simulink library "AFCToolbox"  (R2025b)
settings: Solver=VariableStepAuto  StartTime=0.0  StopTime=10.0  RelTol=1e-3
undefined symbols (not defined in the file or in its folder): AFC5Toolbox_SimuMoudle, ax, ay, az, C_d, C_dm, C_m, C_t, Control, d, declination_table, dp0, dp1, dp2, dp3, dt, euler_0, g0, I_xyz, inclination_table, J_m, lmd_high, lmd_low, lp_acc_knoise, lp_acc_max, lp_acc_min, lp_acc_seed, lp_GPS_BL_max, lp_GPS_BL_min, lp_GPS_H_max, lp_GPS_H_min, lp_GPS_knoise, lp_GPS_seed, lp_GPS_vel_max, lp_GPS_vel_min, lp_gyro_knoise, lp_gyro_max, lp_gyro_min, lp_gyro_seed, lp_hf_vwind, lp_hs_vwind_interp, lp_kaerorho, lp_kaeroT, lp_kIxyz, lp_kmass, lp_momentx_A0, lp_momentx_Af, lp_momentx_ts, lp_momenty_A0, lp_momenty_Af, lp_momenty_ts, lp_momentz_A0, lp_momentz_Af, lp_momentz_ts, lp_vf_vwind, lp_vs_vwind_interp, lp_vwind_thetax, lp_vwind_thetaz, mass, MB_states ... (+52)
libraries: $bdroot x104, simulink x75, etargetslib x32, sharedtransform x13, simulink_extras x12, dspstat3 x11, aerolibconvert2 x9, aerolibtransform2 x3, aerolibutil x2, matrix_library x1
(part 3 of 11)

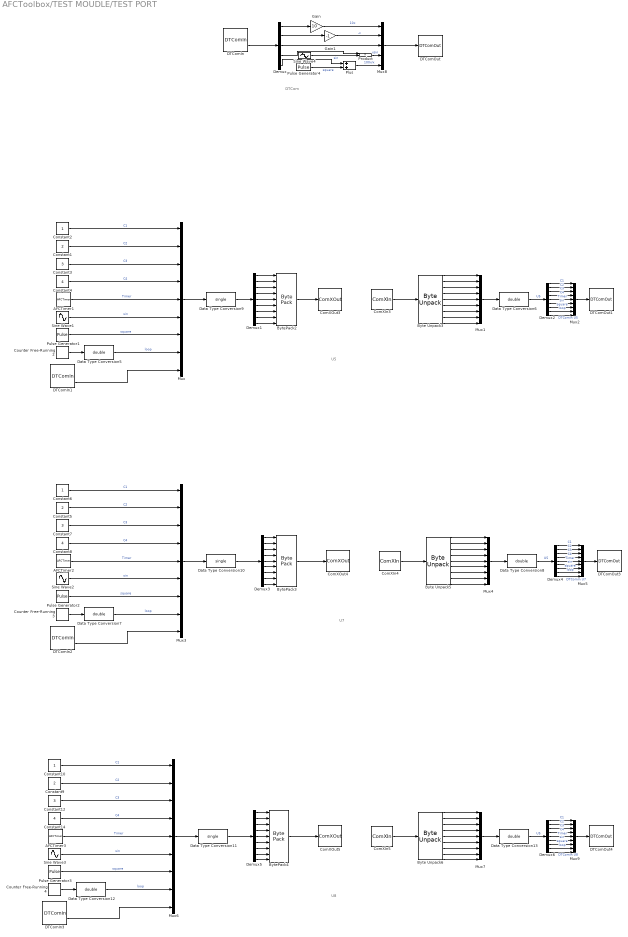
== system AFCToolbox/TEST MOUDLE/TEST PORT ==
  note: U8
  note: DTCom
  note: U7
  note: U5
  AFCTimer1 : $bdroot/DeviceModule/AFCTimer  Priority=0  g_sampleTime=0.002  g_comPort=6  g_instName=0  g_id=0
  AFCTimer2 : $bdroot/DeviceModule/AFCTimer  Priority=0  g_sampleTime=0.002  g_comPort=6  g_instName=0  g_id=0
  AFCTimer3 : $bdroot/DeviceModule/AFCTimer  Priority=0  g_sampleTime=0.002  g_comPort=6  g_instName=0  g_id=0
  Byte Unpack3 : etargetslib/Byte Unpack  dimensions={1,1,1,1,1,1,1,1,1}  datatypes={'single','single','single','single','single','single','single','single','single'}  byteAlign=1
      settings: LibrarySourceBlock=embeddedtargetslib/Host Communication/Byte Unpack
  Byte Unpack5 : etargetslib/Byte Unpack  dimensions={1,1,1,1,1,1,1,1,1}  datatypes={'single','single','single','single','single','single','single','single','single'}  byteAlign=1
      settings: LibrarySourceBlock=embeddedtargetslib/Host Communication/Byte Unpack
  Byte Unpack6 : etargetslib/Byte Unpack  dimensions={1,1,1,1,1,1,1,1,1}  datatypes={'single','single','single','single','single','single','single','single','single'}  byteAlign=1
      settings: LibrarySourceBlock=embeddedtargetslib/Host Communication/Byte Unpack
  BytePack2 : etargetslib/Byte Pack  datatypes={'single','single','single','single','single','single','single','single','single'}  byteAlign=1
  BytePack3 : etargetslib/Byte Pack  datatypes={'single','single','single','single','single','single','single','single','single'}  byteAlign=1
  BytePack4 : etargetslib/Byte Pack  datatypes={'single','single','single','single','single','single','single','single','single'}  byteAlign=1
  ComXIn3 : $bdroot/DeviceModule/ComXIn  Priority=2  g_sampleTime=0.002  g_comPort=UART5(RS422)  g_baudRate=460800  g_dataSize=36  g_parity=0  g_stopBits=1
  ComXIn4 : $bdroot/DeviceModule/ComXIn  Priority=2  g_sampleTime=0.002  g_comPort=UART7(RS232)  g_baudRate=460800  g_dataSize=36  g_parity=0  g_stopBits=1
  ComXIn5 : $bdroot/DeviceModule/ComXIn  Priority=2  g_sampleTime=0.002  g_comPort=UART8(RS232)  g_baudRate=460800  g_dataSize=36  g_parity=0  g_stopBits=1
  ComXOut3 : $bdroot/DeviceModule/ComXOut  Priority=8  g_comPort=UART5(RS422)  g_baudRate=460800  g_outFreq=10
  ComXOut4 : $bdroot/DeviceModule/ComXOut  Priority=8  g_comPort=UART7(RS232)  g_baudRate=460800  g_outFreq=10
  ComXOut5 : $bdroot/DeviceModule/ComXOut  Priority=8  g_comPort=UART8(RS232)  g_baudRate=460800  g_outFreq=10
  Constant1 : Constant  Value=2
  Constant10 : Constant
  Constant12 : Constant  Value=3
  Constant14 : Constant  Value=4
  Constant2 : Constant
  Constant3 : Constant  Value=3
  Constant4 : Constant  Value=4
  Constant5 : Constant  Value=2
  Constant6 : Constant
  Constant7 : Constant  Value=3
  Constant8 : Constant  Value=4
  Constant9 : Constant  Value=2
  Counter Free-Running2 : simulink/Sources/Counter Free-Running  NumBits=8  tsamp=-1
  Counter Free-Running3 : simulink/Sources/Counter Free-Running  NumBits=8  tsamp=-1
  Counter Free-Running4 : simulink/Sources/Counter Free-Running  NumBits=8  tsamp=-1
  DTComIn : $bdroot/DeviceModule/DTComIn  Priority=2  g_sampleTime=0.01  g_frameType=20  g_resFrameNum=0  g_comPort=6  g_instName=0  g_id=0
  DTComIn1 : $bdroot/DeviceModule/DTComIn  Priority=2  g_sampleTime=0.01  g_frameType=25  g_resFrameNum=0  g_comPort=6  g_instName=0  g_id=0
  DTComIn2 : $bdroot/DeviceModule/DTComIn  Priority=2  g_sampleTime=0.01  g_frameType=27  g_resFrameNum=0  g_comPort=6  g_instName=0  g_id=0
  DTComIn3 : $bdroot/DeviceModule/DTComIn  Priority=2  g_sampleTime=0.01  g_frameType=28  g_resFrameNum=0  g_comPort=6  g_instName=0  g_id=0
  DTComOut : $bdroot/DeviceModule/DTComOut  Priority=8  g_frameType=31  g_outFreq=1  g_comPort=0  g_instName=0  g_id=0
  DTComOut1 : $bdroot/DeviceModule/DTComOut  Priority=8  g_frameType=5  g_outFreq=10  g_comPort=0  g_instName=0  g_id=0
  DTComOut3 : $bdroot/DeviceModule/DTComOut  Priority=8  g_frameType=7  g_outFreq=10  g_comPort=0  g_instName=0  g_id=0
  DTComOut4 : $bdroot/DeviceModule/DTComOut  Priority=8  g_frameType=8  g_outFreq=10  g_comPort=0  g_instName=0  g_id=0
  Data Type Conversion10 : DataTypeConversion  OutDataTypeStr=single  SaturateOnIntegerOverflow=off  RndMeth=Floor
  Data Type Conversion11 : DataTypeConversion  OutDataTypeStr=single  SaturateOnIntegerOverflow=off  RndMeth=Floor
  Data Type Conversion{5..8,12..13} (6 alike) : DataTypeConversion  OutDataTypeStr=double  SaturateOnIntegerOverflow=off  RndMeth=Floor
  Data Type Conversion9 : DataTypeConversion  OutDataTypeStr=single  SaturateOnIntegerOverflow=off  RndMeth=Floor
  Demux : Demux  Outputs=5
  Demux{1..6} (6 alike) : Demux  Outputs=9
  Gain : Gain  Gain=10
  Gain1 : Gain  Gain=-1
  Mux{,1..7,9} (9 alike) : Mux  Inputs=9
  Mux8 : Mux  Inputs=5
  Plus : Sum
  Product : Product
  Pulse Generator{1..4} (4 alike) : DiscretePulseGenerator  PulseType=Time based  Amplitude=100  Period=1  PulseWidth=50
  Sine Wave{1..4} (4 alike) : Sin  SineType=Sample based  Samples=100  SampleTime=0.002
  wires:
  Byte Unpack6/8 -> Mux7/8
  Plus/1 -> Mux8/5  "100x/x"
  Demux6/4 -> Mux9/4  "C4"
  Data Type Conversion10/1 -> Demux3/1
  Demux/4 -> Product/1
  Demux6/6 -> Mux9/6  "sin"
  Demux3/3 -> BytePack3/3
  Demux2/9 -> Mux2/9  "DTComIn U5"
  Constant14/1 -> Mux6/4  "C4"
  Demux5/6 -> BytePack4/6
  Demux/5 -> Plus/1
  Gain/1 -> Mux8/1  "10x"
  Demux/1 -> Gain/1
  ComXIn5/1 -> Byte Unpack6/1
  Data Type Conversion13/1 -> Demux6/1  "U5"
  Data Type Conversion8/1 -> Demux4/1  "U5"
  Byte Unpack6/7 -> Mux7/7
  Sine Wave4/1 -> Product/2  "sin"
  AFCTimer1/1 -> Mux/5  "Timer"
  Pulse Generator4/1 -> Plus/2  "square"
  Byte Unpack6/9 -> Mux7/9
  Byte Unpack6/5 -> Mux7/5
  Mux8/1 -> DTComOut/1
  Byte Unpack6/1 -> Mux7/1
  Pulse Generator1/1 -> Mux/7  "square"
  Demux4/6 -> Mux5/6  "sin"
  Byte Unpack6/3 -> Mux7/3
  Byte Unpack5/9 -> Mux4/9
  Byte Unpack5/2 -> Mux4/2
  Demux5/4 -> BytePack4/4
  DTComIn/2 -> Demux/1
  Pulse Generator3/1 -> Mux6/7  "square"
  Byte Unpack3/4 -> Mux1/4
  Demux4/9 -> Mux5/9  "DTComIn U7"
  Demux6/3 -> Mux9/3  "C3"
  Mux4/1 -> Data Type Conversion8/1
  Byte Unpack6/6 -> Mux7/6
  Demux5/7 -> BytePack4/7
  Byte Unpack6/4 -> Mux7/4
  Demux2/7 -> Mux2/7  "square"
  Demux3/9 -> BytePack3/9
  Mux7/1 -> Data Type Conversion13/1
  Demux5/1 -> BytePack4/1
  Demux6/8 -> Mux9/8  "loop"
  Demux1/9 -> BytePack2/9
  Demux3/6 -> BytePack3/6
  Mux9/1 -> DTComOut4/1
  Demux6/1 -> Mux9/1  "C1"
  Demux3/4 -> BytePack3/4
  BytePack4/1 -> ComXOut5/1
  Demux6/9 -> Mux9/9  "DTComIn U8"
  AFCTimer3/1 -> Mux6/5  "Timer"
  Constant12/1 -> Mux6/3  "C3"
  Demux4/7 -> Mux5/7  "square"
  Demux6/5 -> Mux9/5  "Timer"
  Mux6/1 -> Data Type Conversion11/1
  Byte Unpack5/4 -> Mux4/4
  Demux/3 -> Mux8/3
  Demux6/2 -> Mux9/2  "C2"
  Demux2/1 -> Mux2/1  "C1"
  BytePack2/1 -> ComXOut3/1
  Data Type Conversion12/1 -> Mux6/8  "loop"
  Demux3/1 -> BytePack3/1
  Data Type Conversion11/1 -> Demux5/1
  Demux4/5 -> Mux5/5  "Timer"
  Demux3/8 -> BytePack3/8
  Demux5/8 -> BytePack4/8
  Data Type Conversion9/1 -> Demux1/1
  Demux5/5 -> BytePack4/5
  Demux/2 -> Gain1/1
  Demux6/7 -> Mux9/7  "square"
  Gain1/1 -> Mux8/2  "-x"
  Demux5/3 -> BytePack4/3
  Pulse Generator2/1 -> Mux3/7  "square"
  Demux5/2 -> BytePack4/2
  DTComIn3/2 -> Mux6/9
  Demux2/6 -> Mux2/6  "sin"
  Demux2/3 -> Mux2/3  "C3"
  Data Type Conversion6/1 -> Demux2/1  "U5"
  Byte Unpack3/8 -> Mux1/8
  Byte Unpack3/7 -> Mux1/7
  Demux3/7 -> BytePack3/7
  Sine Wave2/1 -> Mux3/6  "sin"
  Constant4/1 -> Mux/4  "C4"
  Demux1/3 -> BytePack2/3
  Demux2/4 -> Mux2/4  "C4"
  DTComIn1/2 -> Mux/9
  Counter Free-Running2/1 -> Data Type Conversion5/1
  Byte Unpack3/2 -> Mux1/2
  Sine Wave1/1 -> Mux/6  "sin"
  Constant2/1 -> Mux/1  "C1"
  Sine Wave3/1 -> Mux6/6  "sin"
  Mux2/1 -> DTComOut1/1
  Byte Unpack3/5 -> Mux1/5
  Byte Unpack3/1 -> Mux1/1
  Demux1/5 -> BytePack2/5
  Mux/1 -> Data Type Conversion9/1
  Byte Unpack3/6 -> Mux1/6
  Mux3/1 -> Data Type Conversion10/1
  Demux1/6 -> BytePack2/6
  ComXIn3/1 -> Byte Unpack3/1
  Byte Unpack3/9 -> Mux1/9
  Constant10/1 -> Mux6/1  "C1"
  Constant6/1 -> Mux3/1  "C1"
  Demux5/9 -> BytePack4/9
  Constant5/1 -> Mux3/2  "C2"
  AFCTimer2/1 -> Mux3/5  "Timer"
  Byte Unpack3/3 -> Mux1/3
  Data Type Conversion7/1 -> Mux3/8  "loop"
  Demux4/1 -> Mux5/1  "C1"
  Demux1/8 -> BytePack2/8
  Constant9/1 -> Mux6/2  "C2"
  Constant1/1 -> Mux/2  "C2"
  Mux1/1 -> Data Type Conversion6/1
  Demux4/4 -> Mux5/4  "C4"
  Demux2/2 -> Mux2/2  "C2"
  Product/1 -> Mux8/4  "xsin"
  DTComIn2/2 -> Mux3/9
  Demux2/8 -> Mux2/8  "loop"
  Demux4/8 -> Mux5/8  "loop"
  Demux3/2 -> BytePack3/2
  Demux1/4 -> BytePack2/4
  ComXIn4/1 -> Byte Unpack5/1
  BytePack3/1 -> ComXOut4/1
  Counter Free-Running3/1 -> Data Type Conversion7/1
  Byte Unpack5/1 -> Mux4/1
  Byte Unpack6/2 -> Mux7/2
  Demux1/1 -> BytePack2/1
  Byte Unpack5/3 -> Mux4/3
  Constant8/1 -> Mux3/4  "C4"
  Demux1/2 -> BytePack2/2
  Demux4/2 -> Mux5/2  "C2"
  Demux4/3 -> Mux5/3  "C3"
  Byte Unpack5/8 -> Mux4/8
  Counter Free-Running4/1 -> Data Type Conversion12/1
  Mux5/1 -> DTComOut3/1
  Constant3/1 -> Mux/3  "C3"
  Byte Unpack5/5 -> Mux4/5
  Byte Unpack5/6 -> Mux4/6
  Data Type Conversion5/1 -> Mux/8  "loop"
  Byte Unpack5/7 -> Mux4/7
  Constant7/1 -> Mux3/3  "C3"
  Demux1/7 -> BytePack2/7
  Demux2/5 -> Mux2/5  "Timer"
  Demux3/5 -> BytePack3/5

== system AFCToolbox/TEST MOUDLE/TEST PORTDOWNLOAD ==
  note: Y
  Data Type Conversion : DataTypeConversion  OutDataTypeStr=boolean  SaturateOnIntegerOverflow=off  RndMeth=Floor
  LedBit : $bdroot/DeviceModule/LedBit  Priority=6  g_chanelNo=黄色指示灯  g_comPort=0  g_instName=0  g_id=0
  Pulse Generator : DiscretePulseGenerator  PulseType=Time based  PulseWidth=50
  wires:
  Pulse Generator/1 -> Data Type Conversion/1
  Data Type Conversion/1 -> LedBit/1

== system AFCToolbox/TEST MOUDLE/TEST PWM ==
  DTComIn1 : $bdroot/DeviceModule/DTComIn  Priority=2  g_sampleTime=0.01  g_frameType=20  g_resFrameNum=0  g_comPort=6  g_instName=0  g_id=0
  DTComIn2 : $bdroot/DeviceModule/DTComIn  Priority=2  Commented=on  g_sampleTime=0.01  g_frameType=20  g_resFrameNum=0  g_comPort=6  g_instName=0  g_id=0
  DTComOut1 : $bdroot/DeviceModule/DTComOut  Priority=8  Commented=on  g_frameType=4  g_outFreq=10  g_comPort=0  g_instName=0  g_id=0
  DTComOut3 : $bdroot/DeviceModule/DTComOut  Priority=8  g_frameType=4  g_outFreq=10  g_comPort=0  g_instName=0  g_id=0
  Demux : Demux  Commented=on  Outputs=2
  Demux1 : Demux  Outputs=12
  HiEscCmd1 : $bdroot/DeviceModule/HiEscCmd  Priority=6  Commented=on  g_chanelNo=2  g_minPW=0  g_maxPW=100  g_comPort=6  g_instName=0  g_id=0
  HiEscCmd10 : $bdroot/DeviceModule/HiEscCmd  Priority=6  g_chanelNo=6  g_minPW=0  g_maxPW=100  g_comPort=6  g_instName=0  g_id=0
  HiEscCmd11 : $bdroot/DeviceModule/HiEscCmd  Priority=6  g_chanelNo=5  g_minPW=0  g_maxPW=100  g_comPort=6  g_instName=0  g_id=0
  HiEscCmd12 : $bdroot/DeviceModule/HiEscCmd  Priority=6  g_chanelNo=4  g_minPW=0  g_maxPW=100  g_comPort=6  g_instName=0  g_id=0
  HiEscCmd13 : $bdroot/DeviceModule/HiEscCmd  Priority=6  g_chanelNo=3  g_minPW=0  g_maxPW=100  g_comPort=6  g_instName=0  g_id=0
  HiEscCmd14 : $bdroot/DeviceModule/HiEscCmd  Priority=6  g_chanelNo=2  g_minPW=0  g_maxPW=100  g_comPort=6  g_instName=0  g_id=0
  HiEscCmd15 : $bdroot/DeviceModule/HiEscCmd  Priority=6  g_chanelNo=1  g_minPW=0  g_maxPW=100  g_comPort=6  g_instName=0  g_id=0
  HiEscCmd2 : $bdroot/DeviceModule/HiEscCmd  Priority=6  Commented=on  g_chanelNo=11  g_minPW=0  g_maxPW=100  g_comPort=6  g_instName=0  g_id=0
  HiEscCmd4 : $bdroot/DeviceModule/HiEscCmd  Priority=6  g_chanelNo=12  g_minPW=0  g_maxPW=100  g_comPort=6  g_instName=0  g_id=0
  HiEscCmd5 : $bdroot/DeviceModule/HiEscCmd  Priority=6  g_chanelNo=11  g_minPW=0  g_maxPW=100  g_comPort=6  g_instName=0  g_id=0
  HiEscCmd6 : $bdroot/DeviceModule/HiEscCmd  Priority=6  g_chanelNo=10  g_minPW=0  g_maxPW=100  g_comPort=6  g_instName=0  g_id=0
  HiEscCmd7 : $bdroot/DeviceModule/HiEscCmd  Priority=6  g_chanelNo=9  g_minPW=0  g_maxPW=100  g_comPort=6  g_instName=0  g_id=0
  HiEscCmd8 : $bdroot/DeviceModule/HiEscCmd  Priority=6  g_chanelNo=8  g_minPW=0  g_maxPW=100  g_comPort=6  g_instName=0  g_id=0
  HiEscCmd9 : $bdroot/DeviceModule/HiEscCmd  Priority=6  g_chanelNo=7  g_minPW=0  g_maxPW=100  g_comPort=6  g_instName=0  g_id=0
  LowEscCmd : $bdroot/DeviceModule/LowEscCmd  Priority=6  Commented=on  g_chanelNo=1  g_minPW=0  g_maxPW=100  g_comPort=6  g_instName=0  g_id=0
  LowEscCmd1 : $bdroot/DeviceModule/LowEscCmd  Priority=6  Commented=on  g_chanelNo=2  g_minPW=0  g_maxPW=100  g_comPort=6  g_instName=0  g_id=0
  LowEscCmd10 : $bdroot/DeviceModule/LowEscCmd  Priority=6  Commented=on  g_chanelNo=11  g_minPW=0  g_maxPW=100  g_comPort=6  g_instName=0  g_id=0
  LowEscCmd11 : $bdroot/DeviceModule/LowEscCmd  Priority=6  Commented=on  g_chanelNo=12  g_minPW=0  g_maxPW=100  g_comPort=6  g_instName=0  g_id=0
  LowEscCmd2 : $bdroot/DeviceModule/LowEscCmd  Priority=6  Commented=on  g_chanelNo=3  g_minPW=0  g_maxPW=100  g_comPort=6  g_instName=0  g_id=0
  LowEscCmd3 : $bdroot/DeviceModule/LowEscCmd  Priority=6  Commented=on  g_chanelNo=4  g_minPW=0  g_maxPW=100  g_comPort=6  g_instName=0  g_id=0
  LowEscCmd4 : $bdroot/DeviceModule/LowEscCmd  Priority=6  Commented=on  g_chanelNo=5  g_minPW=0  g_maxPW=100  g_comPort=6  g_instName=0  g_id=0
  LowEscCmd5 : $bdroot/DeviceModule/LowEscCmd  Priority=6  Commented=on  g_chanelNo=6  g_minPW=0  g_maxPW=100  g_comPort=6  g_instName=0  g_id=0
  LowEscCmd6 : $bdroot/DeviceModule/LowEscCmd  Priority=6  Commented=on  g_chanelNo=7  g_minPW=0  g_maxPW=100  g_comPort=6  g_instName=0  g_id=0
  LowEscCmd7 : $bdroot/DeviceModule/LowEscCmd  Priority=6  Commented=on  g_chanelNo=8  g_minPW=0  g_maxPW=100  g_comPort=6  g_instName=0  g_id=0
  LowEscCmd8 : $bdroot/DeviceModule/LowEscCmd  Priority=6  Commented=on  g_chanelNo=9  g_minPW=0  g_maxPW=100  g_comPort=6  g_instName=0  g_id=0
  LowEscCmd9 : $bdroot/DeviceModule/LowEscCmd  Priority=6  Commented=on  g_chanelNo=10  g_minPW=0  g_maxPW=100  g_comPort=6  g_instName=0  g_id=0
  Mux : Mux  Inputs=14
  Mux1 : Mux  Commented=on
  PWMSample : $bdroot/DeviceModule/PWMSample  Priority=1  g_sampleTime=0.01  g_comPort=6  g_instName=0  g_id=0
  PWMSample1 : $bdroot/DeviceModule/PWMSample  Priority=1  Commented=on  g_sampleTime=0.01  g_comPort=6  g_instName=0  g_id=0
  wires:
  PWMSample1/2 -> Mux1/4  "PWM_IN2"
  Mux1/1 -> DTComOut1/1
  Demux1/3 -> HiEscCmd13/1, Mux/3  "PWM_OUT3"
  Demux1/9 -> HiEscCmd7/1, Mux/9  "PWM_OUT9"
  Demux1/4 -> HiEscCmd12/1, Mux/4  "PWM_OUT4"
  Demux/2 -> HiEscCmd1/1, Mux1/2  "PWM_OUT12"
  Demux/1 -> HiEscCmd2/1, Mux1/1  "PWM_OUT11"
  PWMSample/2 -> Mux/14  "PWM_IN2"
  PWMSample/1 -> Mux/13  "PWM_IN1"
  Demux1/2 -> HiEscCmd14/1, Mux/2  "PWM_OUT2"
  Demux1/7 -> HiEscCmd9/1, Mux/7  "PWM_OUT7"
  Demux1/1 -> HiEscCmd15/1, Mux/1  "PWM_OUT1"
  Demux1/6 -> HiEscCmd10/1, Mux/6  "PWM_OUT6"
  Demux1/5 -> HiEscCmd11/1, Mux/5  "PWM_OUT5"
  Demux1/11 -> HiEscCmd5/1, Mux/11  "PWM_OUT11"
  Demux1/10 -> HiEscCmd6/1, Mux/10  "PWM_OUT10"
  PWMSample1/1 -> Mux1/3  "PWM_IN1"
  DTComIn1/2 -> Demux1/1
  DTComIn2/2 -> Demux/1
  Mux/1 -> DTComOut3/1
  Demux1/8 -> HiEscCmd8/1, Mux/8  "PWM_OUT8"
  Demux1/12 -> HiEscCmd4/1, Mux/12  "PWM_OUT12"

== system AFCToolbox/TEST MOUDLE/TEST SBUS ==
  note: 遥控器通讯模块
  note: PWMout
  Constant : Constant  Value=40
  Constant1 : Constant  Value=30
  Constant10 : Constant  Value=100
  Constant2 : Constant  Value=50
  Constant3 : Constant  Value=60
  Constant4 : Constant  Value=0
  Constant5 : Constant  Value=10
  Constant6 : Constant  Value=20
  Constant7 : Constant  Value=70
  Constant8 : Constant  Value=80
  Constant9 : Constant  Value=90
  DTComOut5 : $bdroot/DeviceModule/DTComOut  Priority=8  g_frameType=6  g_outFreq=10  g_comPort=0  g_instName=0  g_id=0
  HiEscCmd : $bdroot/DeviceModule/HiEscCmd  Priority=6  g_chanelNo=1  g_minPW=40  g_maxPW=80  g_comPort=6  g_instName=0  g_id=0
  HiEscCmd1 : $bdroot/DeviceModule/HiEscCmd  Priority=6  g_chanelNo=9  g_minPW=40  g_maxPW=80  g_comPort=6  g_instName=0  g_id=0
  HiEscCmd2 : $bdroot/DeviceModule/HiEscCmd  Priority=6  g_chanelNo=7  g_minPW=40  g_maxPW=80  g_comPort=6  g_instName=0  g_id=0
  HiEscCmd3 : $bdroot/DeviceModule/HiEscCmd  Priority=6  g_chanelNo=2  g_minPW=40  g_maxPW=80  g_comPort=6  g_instName=0  g_id=0
  Mux1 : Mux  Inputs=10
  SBusCmd : $bdroot/DeviceModule/SBusCmd  Priority=0  g_sampleTime=0.002  g_chanelNo=6  g_comPort=6  g_instName=0  g_id=0
  SBusCmd1 : $bdroot/DeviceModule/SBusCmd  Priority=0  g_sampleTime=0.002  g_chanelNo=1  g_comPort=6  g_instName=0  g_id=0
  SBusCmd2 : $bdroot/DeviceModule/SBusCmd  Priority=0  g_sampleTime=0.002  g_chanelNo=7  g_comPort=6  g_instName=0  g_id=0
  SBusCmd3 : $bdroot/DeviceModule/SBusCmd  Priority=0  g_sampleTime=0.002  g_chanelNo=2  g_comPort=6  g_instName=0  g_id=0
  SBusCmd4 : $bdroot/DeviceModule/SBusCmd  Priority=0  g_sampleTime=0.002  g_chanelNo=9  g_comPort=6  g_instName=0  g_id=0
  SBusCmd5 : $bdroot/DeviceModule/SBusCmd  Priority=0  g_sampleTime=0.002  g_chanelNo=3  g_comPort=6  g_instName=0  g_id=0
  SBusCmd6 : $bdroot/DeviceModule/SBusCmd  Priority=0  g_sampleTime=0.002  g_chanelNo=8  g_comPort=6  g_instName=0  g_id=0
  SBusCmd7 : $bdroot/DeviceModule/SBusCmd  Priority=0  g_sampleTime=0.002  g_chanelNo=4  g_comPort=6  g_instName=0  g_id=0
  SBusCmd8 : $bdroot/DeviceModule/SBusCmd  Priority=0  g_sampleTime=0.002  g_chanelNo=5  g_comPort=6  g_instName=0  g_id=0
  Switch{,2,5,7,9} (5 alike) : Switch  Criteria=u2 > Threshold  Threshold=1600  SaturateOnIntegerOverflow=off  InputSameDT=off
  Switch{1,3..4,6,8} (5 alike) : Switch  Criteria=u2 > Threshold  Threshold=500  SaturateOnIntegerOverflow=off  InputSameDT=off
  wires:
  Constant8/1 -> Switch7/1
  SBusCmd7/1 -> Mux1/10  "Channel4"
  Switch3/1 -> Switch/3
  SBusCmd3/1 -> Mux1/8  "Channel2"
  Switch1/1 -> Switch2/3
  SBusCmd5/1 -> Mux1/9  "Channel3"
  Constant9/1 -> Switch8/1
  Mux1/1 -> DTComOut5/1
  Switch8/1 -> Switch9/3  "pwm4"
  SBusCmd8/1 -> Mux1/1, Switch5/2, Switch4/2  "Channel5"
  Switch2/1 -> Switch6/3  "pwm4"
  SBusCmd4/1 -> Mux1/5, Switch9/2, Switch8/2  "Channel9"
  Constant6/1 -> Switch5/1
  Constant4/1 -> Switch4/3
  Switch4/1 -> Switch5/3
  Constant10/1 -> Switch9/1
  SBusCmd6/1 -> Mux1/4, Switch7/2, Switch6/2  "Channel8"
  Switch5/1 -> Switch3/3
  Constant/1 -> Switch/1
  Switch6/1 -> Switch7/3  "pwm4"
  SBusCmd1/1 -> Mux1/7  "Channel1"
  Switch/1 -> Switch1/3
  Switch9/1 -> Mux1/6, HiEscCmd/1, HiEscCmd1/1, HiEscCmd3/1, HiEscCmd2/1  "PWM"
  SBusCmd/1 -> Mux1/2, Switch/2, Switch3/2  "Channel6"
  Switch7/1 -> Switch8/3  "pwm4"
  SBusCmd2/1 -> Mux1/3, Switch1/2, Switch2/2  "Channel7"
  Constant3/1 -> Switch2/1
  Constant5/1 -> Switch4/1
  Constant1/1 -> Switch3/1
  Constant7/1 -> Switch6/1
  Constant2/1 -> Switch1/1

== system AFCToolbox/TEST MOUDLE/TEST SENSOR ==
  note: 空速计
  note: 磁力计
  note: 气压计
  DPS310 : $bdroot/DeviceModule/DPS310  Priority=1  g_sampleTime=0.01  g_comPort=6  g_instName=0  g_id=0
  DTComOut4 : $bdroot/DeviceModule/DTComOut  Priority=8  g_frameType=2  g_outFreq=10  g_comPort=0  g_instName=0  g_id=0
  IST8310 : $bdroot/DeviceModule/IST8310  Priority=1  g_sampleTime=0.01  g_comPort=0  g_instName=0  g_id=0
  MS5525 : $bdroot/DeviceModule/MS5525  Priority=1  g_sampleTime=0.01  g_comPort=6  g_instName=0  g_id=0
  Mux2 : Mux  Inputs=13
  wires:
  DPS310/1 -> Mux2/6  "Tim"
  DPS310/4 -> Mux2/9  "BarHeight"
  MS5525/2 -> Mux2/11  "IAS_DIFP"
  IST8310/5 -> Mux2/5  "HeadAng"
  IST8310/3 -> Mux2/3  "MagY"
  IST8310/4 -> Mux2/4  "MagZ"
  MS5525/1 -> Mux2/10  "IAS_TIME"
  Mux2/1 -> DTComOut4/1
  IST8310/1 -> Mux2/1  "IST_Tim"
  DPS310/2 -> Mux2/7  "Pressure"
  IST8310/2 -> Mux2/2  "agX"
  DPS310/3 -> Mux2/8  "Temprature"
  MS5525/3 -> Mux2/12  "IAS_TEMP"
  MS5525/4 -> Mux2/13  "IAS"

== system AFCToolbox/TEST MOUDLE/TEST SIMUCOM ==
  DTComOut : $bdroot/DeviceModule/DTComOut  Priority=8  g_frameType=1  g_outFreq=1  g_comPort=0  g_instName=0  g_id=0
  Demux : Demux  Outputs=8
  Mux : Mux  Inputs=8
  SimuComIn : $bdroot/DeviceModule/SimuComIn  Priority=2  g_sampleTime=0.01  g_frameType=80  g_resFrameNum=0  g_comPort=6  g_instName=0  g_id=0
  SimuComOut : $bdroot/DeviceModule/SimuComOut  Priority=8  g_frameType=1  g_outFreq=1  g_comPort=0  g_instName=0  g_id=0
  Terminator3 : Terminator
  wires:
  SimuComIn/2 -> Demux/1, SimuComOut/1
  SimuComIn/1 -> Terminator3/1
  Demux/1 -> Mux/1  "c1"
  Demux/2 -> Mux/2  "c2"
  Demux/3 -> Mux/3  "c3"
  Demux/4 -> Mux/4  "c4"
  Demux/5 -> Mux/5  "timer"
  Demux/6 -> Mux/6  "sin"
  Demux/7 -> Mux/7  "squre"
  Demux/8 -> Mux/8  "loop"
  Mux/1 -> DTComOut/1

== system AFCToolbox/TEST MOUDLE/TEST TDEBUG ==
  Data Type Conversion : DataTypeConversion  OutDataTypeStr=boolean  SaturateOnIntegerOverflow=off  RndMeth=Floor
  LedBit : $bdroot/DeviceModule/LedBit  Priority=6  g_chanelNo=蓝色指示灯  g_comPort=0  g_instName=0  g_id=0
  Pulse Generator : DiscretePulseGenerator  PulseType=Time based  PulseWidth=50
  wires:
  Pulse Generator/1 -> Data Type Conversion/1
  Data Type Conversion/1 -> LedBit/1

== system AFCToolbox/TEST MOUDLE/TSET GPS ==
  note: GPS
  DTComOut : $bdroot/DeviceModule/DTComOut  Priority=8  g_frameType=1  g_outFreq=10  g_comPort=0  g_instName=0  g_id=0
  GPS : $bdroot/DeviceModule/GPS  Priority=1  g_sampleTime=0.1  g_gpsDev=NANO GNSS  g_comPort=6  g_instName=0  g_id=0
  Mux4 : Mux  Inputs=13
  wires:
  GPS/3 -> Mux4/3  "Lat"
  GPS/13 -> Mux4/13  "AFCTim"
  GPS/1 -> Mux4/1  "GPSTim"
  GPS/10 -> Mux4/10  "Sts"
  GPS/9 -> Mux4/9  "Head"
  GPS/12 -> Mux4/12  "hdop"
  GPS/11 -> Mux4/11  "stasN"
  GPS/7 -> Mux4/7  "Vz"
  GPS/6 -> Mux4/6  "Vy"
  Mux4/1 -> DTComOut/1
  GPS/2 -> Mux4/2  "Lon"
  GPS/5 -> Mux4/5  "Vx"
  GPS/8 -> Mux4/8  "Vgnd"
  GPS/4 -> Mux4/4  "Alt"

== system AFCToolbox/基础导航算法模型库/ECL EKF ==
  note: EKF2.cpp -> Run(...)
  note: 2024.03.28午3时半：
      | 整理的新版本EKF导航（single型），包括磁力计、气压计、GPS融合数仿程序
  note: headang
  gyro(rad/s) : Inport
  acc(m2/s) : Inport  Port=2
  Vgps(m/s) : Inport  Port=3
  LLA(deg) : Inport  Port=4
  Gps_sts : Inport  Port=5
  Magxyz(uT) : Inport  Port=6
  BARO_Data(Pa) : Inport  Port=7
  Tim : Inport  Port=8
  Bias Eliminate2 : Subsystem
  Bus Creator : BusCreator  Inputs=q_states(1:4),Vned_states(5:7),Pned_states(8:10),Δθb_states(11:13),ΔVb_states(14:16),MI_states(17:19),MB_states(20:22),Vwind_states(23:24)
  Constant : Constant  Value=[-19.98,-8.18,31.27]
  Data Type Conversion{1,6..8} (4 alike) : DataTypeConversion  OutDataTypeStr=double  SaturateOnIntegerOverflow=off  RndMeth=Floor
  Data Type Conversion{2..5} (4 alike) : DataTypeConversion  OutDataTypeStr=single  SaturateOnIntegerOverflow=off  RndMeth=Floor
  Demux1 : Demux  Outputs=3
  Gain : Gain  Gain=0.01
  Gain10 : Gain  Gain=1/57.3
  Gain11 : Gain  Gain=1/57.3
  Gain12 : Gain
  Gain6 : Gain  Gain=dt
  Gain7 : Gain  Gain=dt
  Gain9 : Gain
  Mux12 : Mux  Inputs=3
  Subsystem : Subsystem
  Subsystem1 : Subsystem
  Subsystem2 : Subsystem
  Subtract : Sum
  Tim1 : InportShadow  Port=8
  Zero-Order Hold10 : ZeroOrderHold  SampleTime=-1
  Zero-Order Hold2 : ZeroOrderHold  SampleTime=dt
  Zero-Order Hold5 : ZeroOrderHold  SampleTime=-1
  Zero-Order Hold8 : ZeroOrderHold  SampleTime=dt
  Zero-Order Hold9 : ZeroOrderHold  SampleTime=-1
  init_state : Subsystem
  states(11:13) : Constant  Value=zeros(1,3)  OutDataTypeStr=single
  states(14:16) : Constant  Value=zeros(1,3)  OutDataTypeStr=single
  states(20:22) : Constant  Value=zeros(1,3)  OutDataTypeStr=single
  states(23:24) : Constant  Value=zeros(1,2)  OutDataTypeStr=single
  ekf_psithephi : Outport
  ekf_xyz : Outport  Port=2
  gps : Outport  Port=3
  Pned : Outport  Port=4
  wires:
  Subtract/1 -> Zero-Order Hold8/1
  Magxyz(uT)/1 -> Subtract/1
  Tim1/1 -> Subsystem1/2(In2)
  Tim/1 -> Subsystem2/2(Tim)
  Demux1/2 -> Gain11/1
  Zero-Order Hold10/1 -> Data Type Conversion5/1
  init_state/3(states(8:10)) -> Bus Creator/3, Data Type Conversion1/1  "Pned_states(8:10)"
  states(14:16)/1 -> Bus Creator/5  "ΔVb_states(14:16)"
  acc(m2/s)/1 -> Zero-Order Hold10/1
  init_state/2(states(5:7)) -> Bus Creator/2  "Vned_states(5:7)"
  states(11:13)/1 -> Bus Creator/4  "Δθb_states(11:13)"
  LLA(deg)/1 -> Data Type Conversion8/1
  Data Type Conversion3/1 -> Bias Eliminate2/1(gyro_B_rad/s_ori)  "gyro_B_rad/s_LPF"
  Zero-Order Hold2/1 -> Data Type Conversion6/1
  Data Type Conversion1/1 -> Pned/1
  init_state/6(Mag_sensordata) -> Subsystem/5(Mag_sensordta)  "Mag_sensordta"
  Subsystem/2(p_ekfnew) -> ekf_xyz/1  "ekf_xyz"
  states(23:24)/1 -> Bus Creator/8  "Vwind_states(23:24)"
  Subsystem/3(GPS_xyz) -> gps/1  "gps"
  Zero-Order Hold5/1 -> init_state/7(baro_data_p)  "BARO_Data"
  Data Type Conversion5/1 -> Gain7/1
  Subsystem/1(ekf_new) -> ekf_psithephi/1  "ekf_psithephi"
  Gain9/1 -> Zero-Order Hold2/1
  Constant/1 -> Subtract/2
  Bias Eliminate2/1(Out1) -> Zero-Order Hold9/1  "gyro_B_rad/s_LPF"
  Vgps(m/s)/1 -> Gain9/1
  Demux1/3 -> Gain12/1
  Data Type Conversion4/1 -> Gain6/1
  Subsystem2/1(enable) -> init_state/6(QGC_sensor_reinit)
  Data Type Conversion8/1 -> Demux1/1
  Subsystem1/1(enable) -> Subsystem/Enable
  Zero-Order Hold8/1 -> Data Type Conversion2/1
  init_state/5(BARO_Data) -> Subsystem/4(BARO_Data)  "BARO_Data"
  Mux12/1 -> init_state/3(gps_LLA_rad)
  Zero-Order Hold9/1 -> Data Type Conversion4/1
  Data Type Conversion2/1 -> Gain/1
  Gain/1 -> init_state/8(mag)  "Guass"
  Data Type Conversion6/1 -> init_state/4(GPS_Vecef_m/s)
  gyro(rad/s)/1 -> Data Type Conversion3/1
  BARO_Data(Pa)/1 -> Zero-Order Hold5/1
  Data Type Conversion7/1 -> init_state/5(GPSfixtype)
  init_state/7(GPS_sensordata) -> Subsystem/6(GPS_sensordata)  "GPS_sensordata"
  Gain10/1 -> Mux12/1
  Gain11/1 -> Mux12/2
  Gain7/1 -> Subsystem/2(imu_delta_vel), init_state/2(imu_data_del_vel)
  Bus Creator/1 -> Subsystem/3(init_states)  "init_states"
  Gain6/1 -> Subsystem/1(imu_delta_angle), init_state/1(imu_delta_ang)
  ? -> init_state/9(states)
  Demux1/1 -> Gain10/1
  init_state/4(states(17:19)) -> Bus Creator/6  "MI_states(17:19)"
  init_state/1(states(1:4)) -> Bus Creator/1  "q_states(1:4)"
  states(20:22)/1 -> Bus Creator/7  "MB_states(20:22)"
  Gain12/1 -> Mux12/3
  Gps_sts/1 -> Subsystem1/1(Gps_sts), Data Type Conversion7/1, Subsystem2/1(Gps_sts)

== system AFCToolbox/ServoCardModule/XSimPack/ByteCheckSum ==
  In1 : Inport
  Add : Sum
  Bitwise AND : simulink/Logic and Bit Operations/Bitwise Operator  logicop=AND  UseBitMask=on  BitMask=hex2dec('FF')  BitMaskRealWorld=Stored Integer
      settings: LibrarySourceBlock=|
      | simulink/Quick Insert/Logic and Bit
      | Operations/Bitwise AND
  Bitwise AND1 : simulink/Logic and Bit Operations/Bitwise Operator  logicop=AND  UseBitMask=on  BitMask=hex2dec('FF')  BitMaskRealWorld=Stored Integer
      settings: LibrarySourceBlock=|
      | simulink/Quick Insert/Logic and Bit
      | Operations/Bitwise AND
  Bitwise NOT : simulink/Logic and Bit Operations/Bitwise Operator  logicop=NOT  UseBitMask=off  BitMask=bin2dec('11011001')  BitMaskRealWorld=Stored Integer
      settings: LibrarySourceBlock=|
      | simulink/Quick Insert/Logic and Bit
      | Operations/Bitwise NOT
  Constant5 : Constant
  Data Type Conversion10 : DataTypeConversion  OutDataTypeStr=uint8  SaturateOnIntegerOverflow=off  RndMeth=Floor
  Data Type Conversion11 : DataTypeConversion  OutDataTypeStr=uint16  SaturateOnIntegerOverflow=off  RndMeth=Floor
  Data Type Conversion12 : DataTypeConversion  OutDataTypeStr=uint8  SaturateOnIntegerOverflow=off  RndMeth=Floor
  Data Type Conversion8 : DataTypeConversion  OutDataTypeStr=uint32  SaturateOnIntegerOverflow=off  RndMeth=Floor
  Data Type Conversion9 : DataTypeConversion  OutDataTypeStr=uint16  SaturateOnIntegerOverflow=off  RndMeth=Floor
  Sum of Elements : Sum  Inputs=+
  Out1 : Outport
  wires:
  Bitwise NOT/1 -> Data Type Conversion9/1
  Constant5/1 -> Data Type Conversion11/1
  Sum of Elements/1 -> Bitwise AND/1
  Bitwise AND/1 -> Data Type Conversion10/1
  Add/1 -> Bitwise AND1/1
  Data Type Conversion9/1 -> Add/1
  Data Type Conversion11/1 -> Add/2
  Data Type Conversion8/1 -> Sum of Elements/1
  Data Type Conversion10/1 -> Bitwise NOT/1
  In1/1 -> Data Type Conversion8/1
  Data Type Conversion12/1 -> Out1/1
  Bitwise AND1/1 -> Data Type Conversion12/1

== system AFCToolbox/ServoCardModule/XSimUnPack/FrameCheck ==
  note: 判断前两个字节帧头、次两个字节帧长度、校验和
  In1 : Inport
  AND : Logic  Inputs=3  IconShape=distinctive  AllPortsSameDT=off  OutDataTypeStr=boolean
  Bitwise AND : simulink/Logic and Bit Operations/Bitwise Operator  logicop=AND  UseBitMask=on  BitMask=hex2dec('FF')  BitMaskRealWorld=Stored Integer
      settings: LibrarySourceBlock=|
      | simulink/Quick Insert/Logic and Bit
      | Operations/Bitwise AND
  Byte Unpack1 : etargetslib/Byte Unpack  dimensions={1}  datatypes={'uint16'}  byteAlign=1
      settings: LibrarySourceBlock=embeddedtargetslib/Host Communication/Byte Unpack
  Byte Unpack3 : etargetslib/Byte Unpack  dimensions={1}  datatypes={'uint16'}  byteAlign=1
      settings: LibrarySourceBlock=embeddedtargetslib/Host Communication/Byte Unpack
  Compare To Constant : simulink/Logic and Bit Operations/Compare To Constant  relop===  const=hex2dec('DAA5')  OutDataTypeStr=boolean
  Compare To Zero : simulink/Logic and Bit Operations/Compare To Zero  relop===  OutDataTypeStr=boolean
  Data Type Conversion : DataTypeConversion  OutDataTypeStr=uint32  SaturateOnIntegerOverflow=off  RndMeth=Floor
  Data Type Conversion1 : DataTypeConversion  OutDataTypeStr=uint8  SaturateOnIntegerOverflow=off  RndMeth=Floor
  Demux : Demux  Outputs=[2,2,-1]
      settings: DisplayOption=none
  Relational Operator : RelationalOperator  Operator===  OutDataTypeStr=boolean  RndMeth=Simplest  InputSameDT=off
  Sum ofElements : Sum  Inputs=+
  Terminator : Terminator
  Width : Width  DataType=uint16
  Out1 : Outport
  wires:
  AND/1 -> Out1/1
  Bitwise AND/1 -> Data Type Conversion1/1
  Demux/1 -> Byte Unpack3/1
  Compare To Constant/1 -> AND/1
  Compare To Zero/1 -> AND/3
  Width/1 -> Relational Operator/2
  Relational Operator/1 -> AND/2
  Demux/2 -> Byte Unpack1/1
  Byte Unpack1/1 -> Relational Operator/1
  In1/1 -> Demux/1, Data Type Conversion/1, Width/1
  Data Type Conversion/1 -> Sum ofElements/1
  Byte Unpack3/1 -> Compare To Constant/1
  Demux/3 -> Terminator/1
  Data Type Conversion1/1 -> Compare To Zero/1
  Sum ofElements/1 -> Bitwise AND/1

== system AFCToolbox/ServoCardModule/XSimUnPack/Subsystem2 ==
  note: 除去帧头等12个字节之外的数据字节长度，如果为4的倍数则正常并解析为单精度，否则不进行解析（强行解析后报错）
  Frame : Inport
  Enable : EnablePort
  Byte Unpack3 : etargetslib/Byte Unpack  dimensions={1}  datatypes={'uint32'}  byteAlign=1
      settings: LibrarySourceBlock=embeddedtargetslib/Host Communication/Byte Unpack
  Compare To Zero : simulink/Logic and Bit Operations/Compare To Zero  relop===  OutDataTypeStr=boolean
  Constant : Constant  Value=4  OutDataTypeStr=uint16
  Data Type Conversion{,1..4} (5 alike) : DataTypeConversion  OutDataTypeStr=double  SaturateOnIntegerOverflow=off  RndMeth=Floor
  Demux : Demux  Outputs=[2,2,4,1,1,1,-1,1]
      settings: DisplayOption=none
  Mod : Math  Operator=mod
  Subsystem : Subsystem
  Terminator : Terminator
  Terminator1 : Terminator
  Terminator2 : Terminator
  Width : Width  DataType=uint16
  FrameCounter : Outport
  SourceID : Outport  Port=2
  TargetID : Outport  Port=3
  FrameType : Outport  Port=4
  FramePara : Outport  Port=5
  wires:
  Constant/1 -> Mod/2
  Data Type Conversion3/1 -> TargetID/1
  Demux/4 -> Data Type Conversion2/1
  Frame/1 -> Demux/1
  Demux/8 -> Terminator/1
  Width/1 -> Mod/1
  Byte Unpack3/1 -> Data Type Conversion1/1
  Demux/3 -> Byte Unpack3/1
  Data Type Conversion4/1 -> FrameType/1
  Data Type Conversion1/1 -> FrameCounter/1
  Demux/6 -> Data Type Conversion4/1
  Demux/5 -> Data Type Conversion3/1
  Demux/2 -> Terminator1/1
  Demux/7 -> Subsystem/1(In1), Width/1
  Data Type Conversion2/1 -> SourceID/1
  Demux/1 -> Terminator2/1
  Subsystem/1(Out1) -> Data Type Conversion/1
  Data Type Conversion/1 -> FramePara/1
  Mod/1 -> Compare To Zero/1
  Compare To Zero/1 -> Subsystem/Enable

== system AFCToolbox/ServoCardModule/XSrvoCmd/查询四个舵机角度指令 ==
  note: 查询四个舵机的角度信息
  note: 长度
  note: 读取数据长度
  Bitwise AND : simulink/Logic and Bit Operations/Bitwise Operator  logicop=AND  UseBitMask=on  BitMask=0xFF  BitMaskRealWorld=Stored Integer
      settings: LibrarySourceBlock=|
      | simulink/Quick Insert/Logic and Bit
      | Operations/Bitwise AND
  Bitwise NOT : simulink/Logic and Bit Operations/Bitwise Operator  logicop=NOT  UseBitMask=off  BitMask=bin2dec('11011001')  BitMaskRealWorld=Stored Integer
      settings: LibrarySourceBlock=|
      | simulink/Quick Insert/Logic and Bit
      | Operations/Bitwise NOT
  Constant10 : Constant  Value=0x38  OutDataTypeStr=uint8
  Constant11 : Constant  Value=0x02  OutDataTypeStr=uint8
  Constant12 : Constant  Value=0xFF  OutDataTypeStr=uint8
  Constant13 : Constant  Value=0x01
  Constant14 : Constant  Value=0x03
  Constant15 : Constant  Value=0x02
  Constant16 : Constant  Value=0x04
  Constant17 : Constant  Value=0x08  OutDataTypeStr=uint8
  Constant6 : Constant  Value=0xFF  OutDataTypeStr=uint8
  Constant7 : Constant  Value=0xFE  OutDataTypeStr=uint8
  Constant9 : Constant  Value=0x82  OutDataTypeStr=uint8
  Data Type Conversion : DataTypeConversion  OutDataTypeStr=uint32  SaturateOnIntegerOverflow=off  RndMeth=Floor
  Data Type Conversion1 : DataTypeConversion  OutDataTypeStr=uint8  SaturateOnIntegerOverflow=off  RndMeth=Floor
  Mux2 : Mux
  Mux3 : Mux  Inputs=9
  Sum ofElements : Sum  Inputs=+
  RAng : Outport
  wires:
  Constant16/1 -> Mux3/9
  Mux3/1 -> Data Type Conversion/1, Mux2/3
  Bitwise AND/1 -> Data Type Conversion1/1
  Data Type Conversion1/1 -> Bitwise NOT/1
  Constant17/1 -> Mux3/2
  Mux2/1 -> RAng/1
  Constant12/1 -> Mux2/2
  Data Type Conversion/1 -> Sum ofElements/1
  Sum ofElements/1 -> Bitwise AND/1
  Constant14/1 -> Mux3/8
  Constant6/1 -> Mux2/1
  Constant13/1 -> Mux3/6
  Constant15/1 -> Mux3/7
  Constant10/1 -> Mux3/4
  Constant11/1 -> Mux3/5
  Bitwise NOT/1 -> Mux2/4
  Constant7/1 -> Mux3/1
  Constant9/1 -> Mux3/3

== system AFCToolbox/ServoCardModule/XSrvoCmd/设置四个舵机位置与速度指令 ==
  Ang : Inport
  Byte Pack : etargetslib/Byte Pack  datatypes={'uint8','uint8','uint8','uint8','uint8','uint8','uint8'}  byteAlign=1
  Constant : Constant  Value=0xFF  OutDataTypeStr=uint8
  Constant1 : Constant  Value=0xFF  OutDataTypeStr=uint8
  Constant2 : Constant  Value=0x20  OutDataTypeStr=uint8
  Constant3 : Constant  Value=0x83  OutDataTypeStr=uint8
  Constant4 : Constant  Value=0x2A  OutDataTypeStr=uint8
  Constant5 : Constant  Value=0x06  OutDataTypeStr=uint8
  Constant6 : Constant  Value=180
  Constant8 : Constant  Value=0xFE  OutDataTypeStr=uint8
  Demux : Demux
  GetCheckSum2 : Subsystem
  Mux : Mux  Inputs=2
  Mux1 : Mux  Inputs=5
  Subsystem1 : Subsystem  mask{id=2}
      mask DialogControl ParameterGroupVar Prompt: id
  Subsystem2 : Subsystem  mask{id=3}
      mask DialogControl ParameterGroupVar Prompt: id
  Subsystem3 : Subsystem  mask{id=4}
      mask DialogControl ParameterGroupVar Prompt: id
  Subsystem5 : Subsystem  mask{id=1}
      mask DialogControl ParameterGroupVar Prompt: id
  Subtract{,1..3} (4 alike) : Sum
  Frame : Outport
  wires:
  Mux/1 -> Frame/1
  Constant4/1 -> Byte Pack/6
  Mux1/1 -> Mux/1, GetCheckSum2/1(In1)
  GetCheckSum2/1(Out1) -> Mux/2
  Constant5/1 -> Byte Pack/7
  Constant2/1 -> Byte Pack/4
  Constant1/1 -> Byte Pack/2
  Constant/1 -> Byte Pack/1
  Constant3/1 -> Byte Pack/5
  Constant8/1 -> Byte Pack/3
  Byte Pack/1 -> Mux1/1
  Demux/3 -> Subtract2/1
  Subtract2/1 -> Subsystem2/1(p)
  Subtract3/1 -> Subsystem3/1(p)
  Ang/1 -> Demux/1
  Demux/1 -> Subtract/1
  Constant6/1 -> Subtract3/2, Subtract2/2, Subtract1/2, Subtract/2
  Subtract1/1 -> Subsystem1/1(p)
  Subtract/1 -> Subsystem5/1(p)
  Demux/2 -> Subtract1/1
  Demux/4 -> Subtract3/1
  Subsystem5/1(Out1) -> Mux1/2
  Subsystem1/1(Out1) -> Mux1/3
  Subsystem2/1(Out1) -> Mux1/4
  Subsystem3/1(Out1) -> Mux1/5

== system AFCToolbox/ServoCardModule/XSrvoSamp/SrvoPro ==
  SvoFrame : Inport
  AND1 : Logic  Inputs=4  IconShape=distinctive  AllPortsSameDT=off  OutDataTypeStr=boolean
  Bitwise AND4 : simulink/Logic and Bit Operations/Bitwise Operator  logicop=AND  UseBitMask=on  BitMask=hex2dec('FF')  BitMaskRealWorld=Stored Integer
      settings: LibrarySourceBlock=|
      | simulink/Quick Insert/Logic and Bit
      | Operations/Bitwise AND
  Byte Unpack4 : etargetslib/Byte Unpack  dimensions={[1]}  datatypes={'uint16'}  byteAlign=1
      settings: LibrarySourceBlock=embeddedtargetslib/Host Communication/Byte Unpack
  Compare To Constant1 : simulink/Logic and Bit Operations/Compare To Constant  relop===  const=0xFF  OutDataTypeStr=boolean
  Compare To Constant2 : simulink/Logic and Bit Operations/Compare To Constant  relop===  const=0x00  OutDataTypeStr=boolean
  Compare To Constant8 : simulink/Logic and Bit Operations/Compare To Constant  relop===  const=0xFFFF  OutDataTypeStr=boolean
  Compare To Constant9 : simulink/Logic and Bit Operations/Compare To Constant  relop===  const=0x04  OutDataTypeStr=boolean
  Data Type Conversion8 : DataTypeConversion  OutDataTypeStr=uint32  SaturateOnIntegerOverflow=off  RndMeth=Floor
  Data Type Conversion9 : DataTypeConversion  OutDataTypeStr=uint8  SaturateOnIntegerOverflow=off  RndMeth=Floor
  Demux : Demux  Outputs=[2,1,1,1,2,1]
  Mux : Mux  Inputs=5
  Subsystem : Subsystem
  Sum ofElements4 : Sum  Inputs=+
  ID : Outport
  angleACK : Outport  Port=2
  wires:
  AND1/1 -> Subsystem/Enable
  Demux/6 -> Mux/5  "CHK"
  Subsystem/1(Outport) -> angleACK/1
  Demux/5 -> Subsystem/1(In1), Mux/4  "POS"
  Demux/3 -> Mux/2, Compare To Constant9/1  "LEN"
  Compare To Constant2/1 -> AND1/3
  Demux/2 -> ID/1, Mux/1  "ID"
  Data Type Conversion8/1 -> Sum ofElements4/1
  Compare To Constant9/1 -> AND1/2
  Sum ofElements4/1 -> Bitwise AND4/1
  Demux/4 -> Compare To Constant2/1, Mux/3  "STS"
  Byte Unpack4/1 -> Compare To Constant8/1
  Mux/1 -> Data Type Conversion8/1
  Compare To Constant8/1 -> AND1/1
  Data Type Conversion9/1 -> Compare To Constant1/1
  Bitwise AND4/1 -> Data Type Conversion9/1
  Demux/1 -> Byte Unpack4/1  "FrameHead"
  Compare To Constant1/1 -> AND1/4
  SvoFrame/1 -> Demux/1

== system AFCToolbox/ServoCardModule/XSrvoSamp/SrvoPro1 ==
  SvoFrame : Inport
  AND1 : Logic  Inputs=4  IconShape=distinctive  AllPortsSameDT=off  OutDataTypeStr=boolean
  Bitwise AND4 : simulink/Logic and Bit Operations/Bitwise Operator  logicop=AND  UseBitMask=on  BitMask=hex2dec('FF')  BitMaskRealWorld=Stored Integer
      settings: LibrarySourceBlock=|
      | simulink/Quick Insert/Logic and Bit
      | Operations/Bitwise AND
  Byte Unpack4 : etargetslib/Byte Unpack  dimensions={[1]}  datatypes={'uint16'}  byteAlign=1
      settings: LibrarySourceBlock=embeddedtargetslib/Host Communication/Byte Unpack
  Compare To Constant1 : simulink/Logic and Bit Operations/Compare To Constant  relop===  const=0xFF  OutDataTypeStr=boolean
  Compare To Constant2 : simulink/Logic and Bit Operations/Compare To Constant  relop===  const=0x00  OutDataTypeStr=boolean
  Compare To Constant8 : simulink/Logic and Bit Operations/Compare To Constant  relop===  const=0xFFFF  OutDataTypeStr=boolean
  Compare To Constant9 : simulink/Logic and Bit Operations/Compare To Constant  relop===  const=0x04  OutDataTypeStr=boolean
  Data Type Conversion8 : DataTypeConversion  OutDataTypeStr=uint32  SaturateOnIntegerOverflow=off  RndMeth=Floor
  Data Type Conversion9 : DataTypeConversion  OutDataTypeStr=uint8  SaturateOnIntegerOverflow=off  RndMeth=Floor
  Demux : Demux  Outputs=[2,1,1,1,2,1]
  Mux : Mux  Inputs=5
  Subsystem : Subsystem
  Sum ofElements4 : Sum  Inputs=+
  ID : Outport
  angleACK : Outport  Port=2
  wires:
  AND1/1 -> Subsystem/Enable
  Demux/6 -> Mux/5  "CHK"
  Subsystem/1(Outport) -> angleACK/1
  Demux/5 -> Subsystem/1(In1), Mux/4  "POS"
  Demux/3 -> Mux/2, Compare To Constant9/1  "LEN"
  Compare To Constant2/1 -> AND1/3
  Demux/2 -> ID/1, Mux/1  "ID"
  Data Type Conversion8/1 -> Sum ofElements4/1
  Compare To Constant9/1 -> AND1/2
  Sum ofElements4/1 -> Bitwise AND4/1
  Demux/4 -> Compare To Constant2/1, Mux/3  "STS"
  Byte Unpack4/1 -> Compare To Constant8/1
  Mux/1 -> Data Type Conversion8/1
  Compare To Constant8/1 -> AND1/1
  Data Type Conversion9/1 -> Compare To Constant1/1
  Bitwise AND4/1 -> Data Type Conversion9/1
  Demux/1 -> Byte Unpack4/1  "FrameHead"
  Compare To Constant1/1 -> AND1/4
  SvoFrame/1 -> Demux/1

== system AFCToolbox/ServoCardModule/XSrvoSamp/SrvoPro2 ==
  SvoFrame : Inport
  AND1 : Logic  Inputs=4  IconShape=distinctive  AllPortsSameDT=off  OutDataTypeStr=boolean
  Bitwise AND4 : simulink/Logic and Bit Operations/Bitwise Operator  logicop=AND  UseBitMask=on  BitMask=hex2dec('FF')  BitMaskRealWorld=Stored Integer
      settings: LibrarySourceBlock=|
      | simulink/Quick Insert/Logic and Bit
      | Operations/Bitwise AND
  Byte Unpack4 : etargetslib/Byte Unpack  dimensions={[1]}  datatypes={'uint16'}  byteAlign=1
      settings: LibrarySourceBlock=embeddedtargetslib/Host Communication/Byte Unpack
  Compare To Constant1 : simulink/Logic and Bit Operations/Compare To Constant  relop===  const=0xFF  OutDataTypeStr=boolean
  Compare To Constant2 : simulink/Logic and Bit Operations/Compare To Constant  relop===  const=0x00  OutDataTypeStr=boolean
  Compare To Constant8 : simulink/Logic and Bit Operations/Compare To Constant  relop===  const=0xFFFF  OutDataTypeStr=boolean
  Compare To Constant9 : simulink/Logic and Bit Operations/Compare To Constant  relop===  const=0x04  OutDataTypeStr=boolean
  Data Type Conversion8 : DataTypeConversion  OutDataTypeStr=uint32  SaturateOnIntegerOverflow=off  RndMeth=Floor
  Data Type Conversion9 : DataTypeConversion  OutDataTypeStr=uint8  SaturateOnIntegerOverflow=off  RndMeth=Floor
  Demux : Demux  Outputs=[2,1,1,1,2,1]
  Mux : Mux  Inputs=5
  Subsystem : Subsystem
  Sum ofElements4 : Sum  Inputs=+
  ID : Outport
  angleACK : Outport  Port=2
  wires:
  AND1/1 -> Subsystem/Enable
  Demux/6 -> Mux/5  "CHK"
  Subsystem/1(Outport) -> angleACK/1
  Demux/5 -> Subsystem/1(In1), Mux/4  "POS"
  Demux/3 -> Mux/2, Compare To Constant9/1  "LEN"
  Compare To Constant2/1 -> AND1/3
  Demux/2 -> ID/1, Mux/1  "ID"
  Data Type Conversion8/1 -> Sum ofElements4/1
  Compare To Constant9/1 -> AND1/2
  Sum ofElements4/1 -> Bitwise AND4/1
  Demux/4 -> Compare To Constant2/1, Mux/3  "STS"
  Byte Unpack4/1 -> Compare To Constant8/1
  Mux/1 -> Data Type Conversion8/1
  Compare To Constant8/1 -> AND1/1
  Data Type Conversion9/1 -> Compare To Constant1/1
  Bitwise AND4/1 -> Data Type Conversion9/1
  Demux/1 -> Byte Unpack4/1  "FrameHead"
  Compare To Constant1/1 -> AND1/4
  SvoFrame/1 -> Demux/1

== system AFCToolbox/ServoCardModule/XSrvoSamp/SrvoPro3 ==
  SvoFrame : Inport
  AND1 : Logic  Inputs=4  IconShape=distinctive  AllPortsSameDT=off  OutDataTypeStr=boolean
  Bitwise AND4 : simulink/Logic and Bit Operations/Bitwise Operator  logicop=AND  UseBitMask=on  BitMask=hex2dec('FF')  BitMaskRealWorld=Stored Integer
      settings: LibrarySourceBlock=|
      | simulink/Quick Insert/Logic and Bit
      | Operations/Bitwise AND
  Byte Unpack4 : etargetslib/Byte Unpack  dimensions={[1]}  datatypes={'uint16'}  byteAlign=1
      settings: LibrarySourceBlock=embeddedtargetslib/Host Communication/Byte Unpack
  Compare To Constant1 : simulink/Logic and Bit Operations/Compare To Constant  relop===  const=0xFF  OutDataTypeStr=boolean
  Compare To Constant2 : simulink/Logic and Bit Operations/Compare To Constant  relop===  const=0x00  OutDataTypeStr=boolean
  Compare To Constant8 : simulink/Logic and Bit Operations/Compare To Constant  relop===  const=0xFFFF  OutDataTypeStr=boolean
  Compare To Constant9 : simulink/Logic and Bit Operations/Compare To Constant  relop===  const=0x04  OutDataTypeStr=boolean
  Data Type Conversion8 : DataTypeConversion  OutDataTypeStr=uint32  SaturateOnIntegerOverflow=off  RndMeth=Floor
  Data Type Conversion9 : DataTypeConversion  OutDataTypeStr=uint8  SaturateOnIntegerOverflow=off  RndMeth=Floor
  Demux : Demux  Outputs=[2,1,1,1,2,1]
  Mux : Mux  Inputs=5
  Subsystem : Subsystem
  Sum ofElements4 : Sum  Inputs=+
  ID : Outport
  angleACK : Outport  Port=2
  wires:
  AND1/1 -> Subsystem/Enable
  Demux/6 -> Mux/5  "CHK"
  Subsystem/1(Outport) -> angleACK/1
  Demux/5 -> Subsystem/1(In1), Mux/4  "POS"
  Demux/3 -> Mux/2, Compare To Constant9/1  "LEN"
  Compare To Constant2/1 -> AND1/3
  Demux/2 -> ID/1, Mux/1  "ID"
  Data Type Conversion8/1 -> Sum ofElements4/1
  Compare To Constant9/1 -> AND1/2
  Sum ofElements4/1 -> Bitwise AND4/1
  Demux/4 -> Compare To Constant2/1, Mux/3  "STS"
  Byte Unpack4/1 -> Compare To Constant8/1
  Mux/1 -> Data Type Conversion8/1
  Compare To Constant8/1 -> AND1/1
  Data Type Conversion9/1 -> Compare To Constant1/1
  Bitwise AND4/1 -> Data Type Conversion9/1
  Demux/1 -> Byte Unpack4/1  "FrameHead"
  Compare To Constant1/1 -> AND1/4
  SvoFrame/1 -> Demux/1

== system AFCToolbox/SimuMoudle/Equations of Motion1/NED2LLA ==
  lat(deg) : Inport
  lon(deg) : Inport  Port=2
  h(m) : Inport  Port=3
  N : Inport  Port=4
  U : Inport  Port=5
  E : Inport  Port=6
  Add : Sum
  Demux : Demux  Outputs=2
  Direction Cosine Matrix ECEF to NED : aerolibtransform2/Direction Cosine Matrix ECEF to NED
  ECEF Position to LLA1 : ECEF2LLA  R=6378137
  Gain : Gain  Gain=-1
  LLA to ECEF Position : LLA2ECEF  R=6378137
  Mux : Mux  Inputs=2
  Mux1 : Mux  Inputs=3
  Product : Product  Multiplication=Matrix(*)
  Transpose : Math  Operator=transpose  SignedPower=on
  latout(deg) : Outport
  lonout(deg) : Outport  Port=2
  altout(m) : Outport  Port=3
  wires:
  LLA to ECEF Position/1 -> Add/1
  Transpose/1 -> Product/1
  Direction Cosine Matrix ECEF to NED/1 -> Transpose/1
  h(m)/1 -> LLA to ECEF Position/2
  Add/1 -> ECEF Position to LLA1/1
  Product/1 -> Add/2
  ECEF Position to LLA1/2 -> altout(m)/1
  lat(deg)/1 -> Mux/1
  lon(deg)/1 -> Mux/2
  Mux/1 -> Direction Cosine Matrix ECEF to NED/1, LLA to ECEF Position/1
  ECEF Position to LLA1/1 -> Demux/1
  Demux/1 -> latout(deg)/1
  Demux/2 -> lonout(deg)/1
  U/1 -> Gain/1
  N/1 -> Mux1/1
  E/1 -> Mux1/2
  Gain/1 -> Mux1/3
  Mux1/1 -> Product/2

== system AFCToolbox/SimuMoudle/Equations of Motion1/w x ( I w ) ==
  a(1) a(2) a(3) : Inport
  b(1) b(2) b(3) : Inport  Port=2
  Product : Product  RndMeth=Zero
  Product1 : Product  RndMeth=Zero
  Selector : Selector  InputPortWidth=3  IndexOptions=Index vector (dialog)  Indices=[2 3 1]  OutputSizes=1
  Selector1 : Selector  InputPortWidth=3  IndexOptions=Index vector (dialog)  Indices=[3 1 2]  OutputSizes=1
  Selector2 : Selector  InputPortWidth=3  IndexOptions=Index vector (dialog)  Indices=[3 1 2]  OutputSizes=1
  Selector3 : Selector  InputPortWidth=3  IndexOptions=Index vector (dialog)  Indices=[2 3 1]  OutputSizes=1
  Sum : Sum  Inputs=+|-
  c(1) c(2) c(3) : Outport
  wires:
  b(1) b(2) b(3)/1 -> Selector2/1, Selector3/1
  a(1) a(2) a(3)/1 -> Selector1/1, Selector/1
  Selector2/1 -> Product/2
  Selector1/1 -> Product1/1
  Selector3/1 -> Product1/2
  Selector/1 -> Product/1
  Sum/1 -> c(1) c(2) c(3)/1
  Product1/1 -> Sum/2
  Product/1 -> Sum/1

== system AFCToolbox/SimuMoudle/Forces & Moments1/Forces ==
  B to G : Inport
  w1234 : Inport  Port=2
  Vb_a : Inport  Port=3
  mass : Inport  Port=4
  g : Inport  Port=5
  Abs : Abs  SaturateOnIntegerOverflow=off
  Constant 0 : Constant  Value=0
  Constant 1 : Constant  Value=0
  Gain : Gain  Gain=C_t
  Gain1 : Gain  Gain=C_d
  Gain2 : Gain  Gain=-1
  Mux : Mux  Inputs=3
  N SD : Scope  Commented=on
      settings: TimeSpan=35  ActiveDisplayYMinimum=-3.0081  ActiveDisplayYMaximum=1.03866  DataLoggingVariableName=SD_ng  DataLoggingSaveFormat=Array
  Product B2G * F : Product  Multiplication=Matrix(*)  RndMeth=Zero
  Product F/G : Product  Inputs=*/  RndMeth=Zero
  Product mg0 : Product  Inputs=**  RndMeth=Zero
  Product mgxyz : Product  Inputs=**  RndMeth=Zero
  Product1 : Product
  Product2 : Product
  Scope : Scope
      settings: ActiveDisplayYMinimum=-113.23371  ActiveDisplayYMaximum=27.21629  DataLoggingVariableName=ScopeData10
  Subsystem : Subsystem
  Sum of Elements : Sum  Inputs=+
  add : Sum  Inputs=2
  add1 : Sum  Inputs=2
  "F " : Outport
  wires:
  Vb_a/1 -> Abs/1, Product2/1
  B to G/1 -> Product B2G * F/1
  Product mgxyz/1 -> add1/2
  add1/1 -> "F "/1
  Product B2G * F/1 -> add1/1
  Product F/G/1 -> N SD/1
  g/1 -> Subsystem/2(g0), Product mg0/2
  mass/1 -> Product mgxyz/1, Product mg0/1
  Subsystem/1(gravity) -> Product mgxyz/2
  Constant 0/1 -> Subsystem/1(Zero)
  Product mg0/1 -> Product F/G/2
  w1234/1 -> Product1/2, Product1/1
  Product1/1 -> Sum of Elements/1
  Sum of Elements/1 -> Gain/1
  Abs/1 -> Product2/2
  Product2/1 -> Gain1/1
  Gain/1 -> Gain2/1
  Constant 1/1 -> Mux/2, Mux/1
  Mux/1 -> add/1
  add/1 -> Scope/1, Product B2G * F/2, Product F/G/1
  Gain2/1 -> Mux/3
  Gain1/1 -> add/2
